simulink model "quartercar_RL_6_no_G_control_input"  (R2023a)
settings: Solver=VariableStepAuto  StartTime=0  StopTime=5  FixedStep=0.0001  RelTol=1e-5  EnableMultiTasking=on
undefined symbols (not defined in the file or in its folder): magnitude
libraries: simulink x2, rllib x1
settings Model: Creator=Administrator  LastModifiedBy=Yuk
settings DataIOCC: SaveFormat=Array
settings OptimizationCC: LifeSpan=inf
settings DebuggingCC: AlgebraicLoopMsg=none  UnderspecifiedInitializationDetection=Classic  MergeDetectMultiDrivingBlocksExec=none  SolverPrmCheckMsg=warning  UnconnectedInputMsg=warning  UnconnectedOutputMsg=warning  UnconnectedLineMsg=warning  StateNameClashWarn=warning  SFUnexpectedBacktrackingDiag=warning  SFNoUnconditionalDefaultTransitionDiag=warning  SFExecutionAtInitializationDiag=none  ArithmeticOperatorsInVariantConditions=warning
settings HardwareCC: ProdBitPerPointer=32  ProdBitPerSizeT=32  ProdBitPerPtrDiffT=32  ProdLargestAtomicFloat=None  ProdIntDivRoundTo=Undefined  ProdEndianess=Unspecified  ProdWordSize=32  ProdHWDeviceType=32-bit Generic
settings ModelReferenceCC: PropagateSignalLabelsOutOfModel=off
settings SFSimCC: SimUseLocalCustomCode=off  CustomCodeUndefinedFunction=UseInterfaceOnly  SimTargetLang=C++
settings RTWCC: RTWUseLocalCustomCode=off
settings CodeAppCC: StateflowObjectComments=on
settings GRTTargetCC: TargetLangStandard=C89/C90 (ANSI)
settings ConfigComp: CovMetricSettings=dw  CovSaveCumulativeToWorkspaceVar=on  CovSaveSingleToWorkspaceVar=on  CovExternalEMLEnable=off

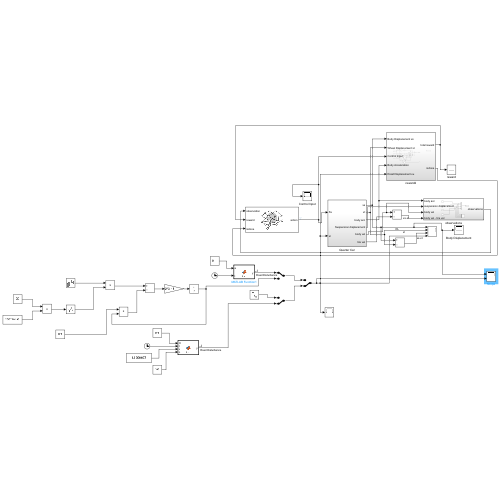
[thumbnail: Simulink's stored preview of the top-level diagram]
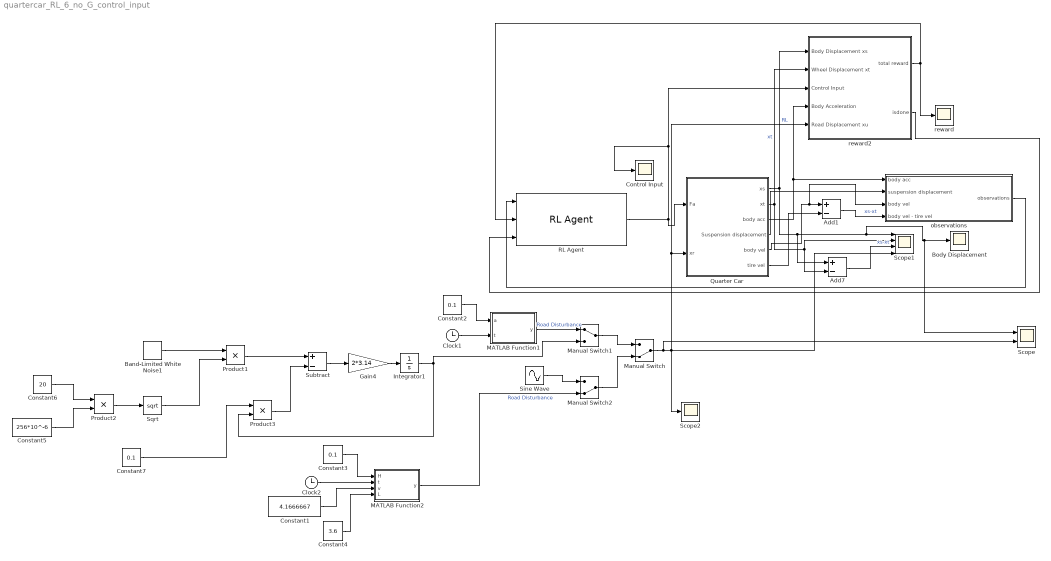
== system quartercar_RL_6_no_G_control_input ==
  Add1 : Sum  Inputs=+-
  Add7 : Sum  Inputs=+-
  Band-Limited White Noise1 : simulink/Sources/Band-Limited White Noise  Cov=[5.4*10^-3]  Ts=0.1  seed=[23341]
  Body Displacement : Scope
  Clock1 : Clock
  Clock2 : Clock
  Constant1 : Constant  Value=4.1666667
  Constant2 : Constant  Value=0.1
  Constant3 : Constant  Value=0.1
  Constant4 : Constant  Value=3.6
  Constant5 : Constant  Value=256*10^-6
  Constant6 : Constant  Value=20
  Constant7 : Constant  Value=0.1
  Control Input : Scope
  Gain4 : Gain  Gain=2*3.14
  Integrator1 : Integrator
  MATLAB Function1 : MATLAB Function  TreatAsAtomicUnit=on
  MATLAB Function2 : MATLAB Function  TreatAsAtomicUnit=on
  Manual Switch : ManualSwitch  CurrentSetting=0
  Manual Switch1 : ManualSwitch
  Manual Switch2 : ManualSwitch  CurrentSetting=0
  Product1 : Product
  Product2 : Product
  Product3 : Product
  Quarter Car : Subsystem
  RL Agent : rllib/RL Agent  Agent=agent  ExternalActionAsInput=off  ProvideLastAction=off  ProvideCumRwd=off  TreatAsDirectFeedthrough=on  UseStrictObservationDataTypes=off
  Scope : Scope  NumInputPorts=2
  Scope1 : Scope  NumInputPorts=4
  Scope2 : Scope
  Sine Wave : Sin  Amplitude=0.1  Frequency=0.5  SampleTime=0
  Sqrt : Sqrt
  Subtract : Sum  Inputs=+-
  observations : Subsystem
  reward : Scope
  reward2 : Subsystem
  wires:
  Quarter Car/1(xs) -> reward2/1(Body Displacement xs), Add7/1, Body Displacement/1, Scope/1, Scope1/1  "RL"
  Quarter Car/2(xt) -> Add7/2, Scope1/2, reward2/2(Wheel Displacement xt)  "xt"
  Add7/1 -> Scope1/3  "xs-xt"
  Constant2/1 -> MATLAB Function1/1(a)
  Clock1/1 -> MATLAB Function1/2(t)
  reward2/1(total reward) -> reward/1, RL Agent/2
  Quarter Car/3(body acc) -> reward2/4(Body Acceleration), observations/1(body acc)
  observations/1(observations) -> RL Agent/1
  reward2/2(isdone) -> RL Agent/3
  Quarter Car/4(Suspension displacement) -> observations/2(suspension displacement)
  Quarter Car/5(body vel) -> observations/3(body vel), Add1/1
  Quarter Car/6(tire vel) -> Add1/2
  Add1/1 -> observations/4(body vel - tire vel)  "xs-xt"
  RL Agent/1 -> Quarter Car/1(Fa), Control Input/1, reward2/3(Control Input)
  Manual Switch/1 -> Scope/2, Scope1/4, reward2/5(Road Displacement xu), Quarter Car/2(xr), Scope2/1
  Manual Switch1/1 -> Manual Switch/1
  MATLAB Function1/1(y) -> Manual Switch1/1  "Road Disturbance"
  Integrator1/1 -> Manual Switch1/2, Product3/2
  Constant5/1 -> Product2/2
  Sqrt/1 -> Product1/2
  Constant6/1 -> Product2/1
  Product2/1 -> Sqrt/1
  Constant7/1 -> Product3/1
  Gain4/1 -> Integrator1/1
  Product1/1 -> Subtract/1
  Band-Limited White Noise1/1 -> Product1/1
  Product3/1 -> Subtract/2
  Subtract/1 -> Gain4/1
  MATLAB Function2/1(y) -> Manual Switch2/2  "Road Disturbance"
  Constant1/1 -> MATLAB Function2/3(v)
  Clock2/1 -> MATLAB Function2/2(t)
  Constant3/1 -> MATLAB Function2/1(H)
  Constant4/1 -> MATLAB Function2/4(L)
  Manual Switch2/1 -> Manual Switch/2
  Sine Wave/1 -> Manual Switch2/1

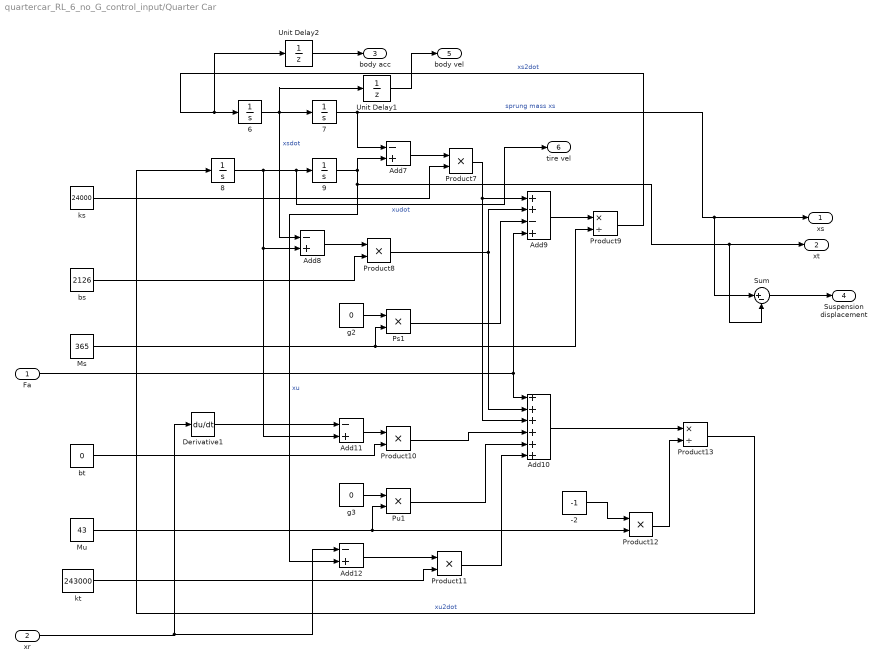
== system quartercar_RL_6_no_G_control_input/Quarter Car ==
  Fa : Inport
  xr : Inport  Port=2
  -2 : Constant  Value=-1
  {6..9} (4 alike) : Integrator
  Add10 : Sum  Inputs=++++++
  Add{7..8,11..12} (4 alike) : Sum  Inputs=-+
  Add9 : Sum  Inputs=++-+
  Derivative1 : Derivative
  Ms : Constant  Value=365
  Mu : Constant  Value=43
  Product{7..8,10..12} (5 alike) : Product
  Product13 : Product  Inputs=*/
  Product9 : Product  Inputs=*/
  Ps1 : Product
  Pu1 : Product
  Sum : Sum  Inputs=|+-
  Unit Delay1 : UnitDelay  SampleTime=-1  HasFrameUpgradeWarning=on
  Unit Delay2 : UnitDelay  SampleTime=-1  HasFrameUpgradeWarning=on
  bs : Constant  Value=2126
  bt : Constant  Value=0
  g2 : Constant  Value=0
  g3 : Constant  Value=0
  ks : Constant  Value=24000
  kt : Constant  Value=243000
  xs : Outport
  xt : Outport  Port=2
  body acc : Outport  Port=3
  Suspension displacement : Outport  Port=4
  body vel : Outport  Port=5
  tire vel : Outport  Port=6
  wires:
  g2/1 -> Ps1/1
  Product12/1 -> Product13/2
  g3/1 -> Pu1/1
  Ps1/1 -> Add9/3
  Add10/1 -> Product13/1
  -2/1 -> Product12/1
  Mu/1 -> Pu1/2, Product12/2
  Product11/1 -> Add10/6
  Add12/1 -> Product11/1
  kt/1 -> Product11/2
  xr/1 -> Add12/1, Derivative1/1
  Pu1/1 -> Add10/5
  Product10/1 -> Add10/4
  Add11/1 -> Product10/1
  bt/1 -> Product10/2
  Derivative1/1 -> Add11/1
  Ms/1 -> Product9/2, Ps1/2
  Add9/1 -> Product9/1
  Fa/1 -> Add10/1, Add9/4
  Product8/1 -> Add10/2, Add9/2
  Product7/1 -> Add10/3, Add9/1
  bs/1 -> Product8/2
  Add8/1 -> Product8/1
  ks/1 -> Product7/2
  Add7/1 -> Product7/1
  9/1 -> Add12/2, Sum/2, xt/1, Add7/2  "xu"
  Product13/1 -> 8/1  "xu2dot"
  8/1 -> tire vel/1, 9/1, Add8/2, Add11/2  "xudot"
  7/1 -> Add7/1, Sum/1, xs/1  "sprung mass xs"
  Product9/1 -> Unit Delay2/1, 6/1  "xs2dot"
  6/1 -> Unit Delay1/1, 7/1, Add8/1  "xsdot"
  Sum/1 -> Suspension displacement/1
  Unit Delay1/1 -> body vel/1
  Unit Delay2/1 -> body acc/1

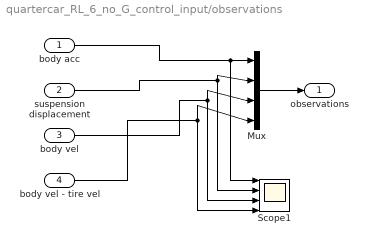
== system quartercar_RL_6_no_G_control_input/observations ==
  body acc : Inport
  suspension displacement : Inport  Port=2
  body vel : Inport  Port=3
  body vel - tire vel : Inport  Port=4
  Mux : Mux
  Scope1 : Scope  NumInputPorts=4
  observations : Outport
  wires:
  body acc/1 -> Scope1/1, Mux/1
  Mux/1 -> observations/1
  body vel/1 -> Scope1/3, Mux/3
  suspension displacement/1 -> Scope1/2, Mux/2
  body vel - tire vel/1 -> Scope1/4, Mux/4

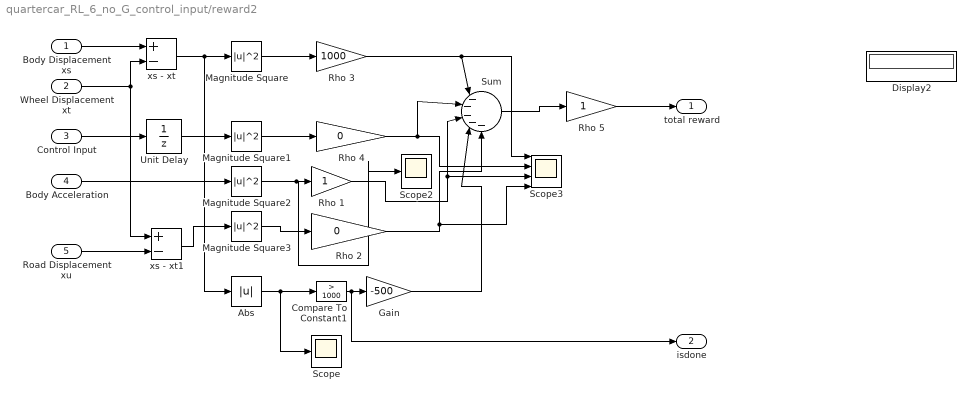
== system quartercar_RL_6_no_G_control_input/reward2 ==
  Body Displacement xs : Inport
  Wheel Displacement xt : Inport  Port=2
  Control Input : Inport  Port=3
  Body Acceleration : Inport  Port=4
  Road Displacement xu : Inport  Port=5
  Abs : Abs  SaturateOnIntegerOverflow=off
  Compare To Constant1 : simulink/Logic and Bit Operations/Compare To Constant  relop=>  const=1000  OutDataTypeStr=boolean
  Display2 : Display
  Gain : Gain  Gain=-500
  Magnitude Square{,1..3} (4 alike) : Math  Operator=magnitude^2  SignedPower=on  RndMeth=Zero
  Rho 1 : Gain
  Rho 2 : Gain  Gain=0
  Rho 3 : Gain  Gain=1000
  Rho 4 : Gain  Gain=0
  Rho 5 : Gain
  Scope : Scope
  Scope2 : Scope
  Scope3 : Scope  NumInputPorts=4
  Sum : Sum  Inputs=|-----
  Unit Delay : UnitDelay  SampleTime=-1  HasFrameUpgradeWarning=on
  xs - xt : Sum  Inputs=+-
  xs - xt1 : Sum  Inputs=+-
  total reward : Outport
  isdone : Outport  Port=2
  wires:
  Wheel Displacement xt/1 -> xs - xt1/1, xs - xt/2
  Body Displacement xs/1 -> xs - xt/1
  Magnitude Square2/1 -> Scope2/1, Rho 1/1
  xs - xt/1 -> Magnitude Square/1, Abs/1
  Magnitude Square/1 -> Rho 3/1
  Control Input/1 -> Unit Delay/1
  Unit Delay/1 -> Magnitude Square1/1
  Rho 3/1 -> Scope3/1, Sum/1
  Compare To Constant1/1 -> isdone/1, Gain/1
  Rho 1/1 -> Scope3/3, Sum/3
  Gain/1 -> Sum/4
  Body Acceleration/1 -> Magnitude Square2/1
  Rho 5/1 -> total reward/1
  Abs/1 -> Scope/1, Compare To Constant1/1
  Rho 4/1 -> Scope3/2, Sum/2
  Magnitude Square1/1 -> Rho 4/1
  Road Displacement xu/1 -> xs - xt1/2
  xs - xt1/1 -> Magnitude Square3/1
  Magnitude Square3/1 -> Rho 2/1
  Rho 2/1 -> Scope3/4, Sum/5
  Sum/1 -> Rho 5/1

== matlab function quartercar_RL_6_no_G_control_input/MATLAB Function2 ==
  data: H input; y output; t input; v input; L input
function y = fcn(H,t,v,L)
% CODE GENERATION
if (1<t) && (t<L/v+1)
    
  y=H/2*(1-cos((2*pi*v/L)*(t-1)));
% w = 2*pi*v/L;
%   y=H*(1-cos(w*t));

else
    y=0;
end
out=y;

== matlab function quartercar_RL_6_no_G_control_input/MATLAB Function1 ==
  data: a input; y output; t input
function y = fcn(a,t)
% CODE GENERATION
if (t>=1 && t<=2)
    
    % y= a*(1-cos(2*pi*t))/2;
    y= 0.1-a/2*(1+cos(2*pi*t));
    % y= a-(a/2*(1-cos(2*pi*t)));
% elseif (t>=5.5 && t<=6.5)
%     y= 0.07/2*(1+cos(2*pi*t));

else
    y=0;
end
out=y;
